simulink model "XROBO02_reference"  (R2025a)
settings: Solver=ode15s  StartTime=0  StopTime=8  MaxStep=0.002  RelTol=1e-3  AbsTol=1e-3
undefined symbols (not defined in the file): cube_l, disturbance_start, disturbance_torque_nm, F1, F2, left_target_rad, move_duration, right_target_rad, shared_payload_mass, torque_limit_scale, X, Y, Z
libraries: sm_lib x210, nesl_utility x45
(part 2 of 5)

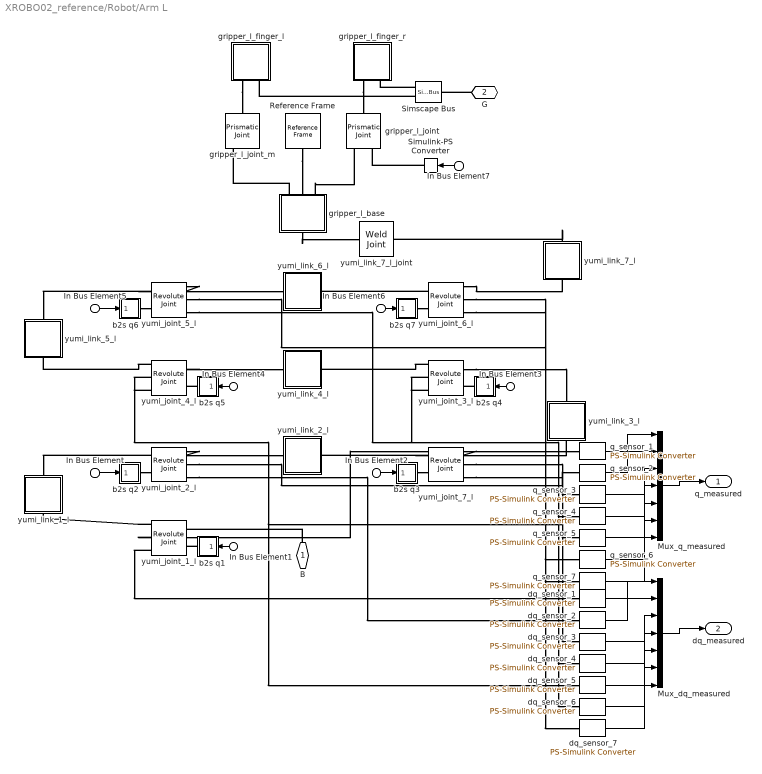
== system XROBO02_reference/Robot/Arm L ==
  In Bus Element1 : Inport  PortName=q  Element=q1
  In Bus Element : Inport  PortName=q  Element=q2
  In Bus Element2 : Inport  PortName=q  Element=q3
  In Bus Element3 : Inport  PortName=q  Element=q4
  In Bus Element4 : Inport  PortName=q  Element=q5
  In Bus Element5 : Inport  PortName=q  Element=q6
  In Bus Element6 : Inport  PortName=q  Element=q7
  In Bus Element7 : Inport  PortName=q  Element=f
  Mux_dq_measured : Mux  Inputs=7
  Mux_q_measured : Mux  Inputs=7
  Reference Frame : sm_lib/Frames and Transforms/Reference Frame
  Simscape Bus : SimscapeBus  HierarchyStrings=F1;F2
  Simulink-PS Converter : nesl_utility/Simulink-PS Converter  PhysicalDomain=network_engine_domain  SubClassName=ps_input  LeftPortType=input  RightPortType=output  PseudoPeriodic=off  Frequencies=[]  NoiseDistribution=none  NoiseParameters=[]  Unit=m  AffineConversion=off  FilteringAndDerivatives=filter  SimscapeFilterOrder=2  InputFilterTimeConstant=0.1  UdotUserProvided=0
  b2s q1 : Subsystem
  b2s q2 : Subsystem
  b2s q3 : Subsystem
  b2s q4 : Subsystem
  b2s q5 : Subsystem
  b2s q6 : Subsystem
  b2s q7 : Subsystem
  dq_sensor_{1..7} (7 alike) : nesl_utility/PS-Simulink Converter  PhysicalDomain=network_engine_domain  SubClassName=ps_output  LeftPortType=input  RightPortType=output  PseudoPeriodic=off  Frequencies=[]  VectorFormat=inherit  Unit=rad/s  AffineConversion=off
  gripper_l_base : Subsystem
  gripper_l_finger_l : Subsystem
  gripper_l_finger_r : Subsystem
  gripper_l_joint : sm_lib/Joints/Prismatic Joint  JointMode=Normal  CompositeWrenchDir=FollowerOnBase  CompositeWrenchFrame=BaseFrame  SenseConstraintForce=off  SenseConstraintTorque=off  SenseTotalForce=off  SenseTotalTorque=off  PositionTargetSpecify=off  PositionTargetPriority=High  PositionTargetValue=0  PositionTargetValueUnits=m  VelocityTargetSpecify=off  VelocityTargetPriority=High  VelocityTargetValue=0  VelocityTargetValueUnits=m/s  EquilibriumPosition=0  EquilibriumPositionUnits=m  SpringStiffness=0  SpringStiffnessUnits=N/m  DampingCoefficient=1  DampingCoefficientUnits=kg/s  LowerLimitSpecify=on  LowerLimitBound=0  LowerLimitBoundUnits=m  LowerLimitStiffness=1e6  LowerLimitStiffnessUnits=N/m  LowerLimitDamping=1e3  LowerLimitDampingUnits=N/(m/s)  LowerLimitTransitionRegionWidth=1e-4  LowerLimitTransitionRegionWidthUnits=m  UpperLimitSpecify=on  UpperLimitBound=0.025  UpperLimitBoundUnits=m  UpperLimitStiffness=1e6  UpperLimitStiffnessUnits=N/m  UpperLimitDamping=1e3  UpperLimitDampingUnits=N/(m/s)  UpperLimitTransitionRegionWidth=1e-4  UpperLimitTransitionRegionWidthUnits=m  TorqueActuationMode=ComputedTorque  MotionActuationMode=InputMotion  SensePosition=off  SenseVelocity=off  SenseAcceleration=off  SenseTorqueForce=off  SenseLowerLimitTorqueForce=off  SenseUpperLimitTorqueForce=off
  gripper_l_joint_m : sm_lib/Joints/Prismatic Joint  JointMode=Normal  CompositeWrenchDir=FollowerOnBase  CompositeWrenchFrame=BaseFrame  SenseConstraintForce=off  SenseConstraintTorque=off  SenseTotalForce=off  SenseTotalTorque=off  PositionTargetSpecify=off  PositionTargetPriority=High  PositionTargetValue=0  PositionTargetValueUnits=m  VelocityTargetSpecify=off  VelocityTargetPriority=High  VelocityTargetValue=0  VelocityTargetValueUnits=m/s  EquilibriumPosition=0  EquilibriumPositionUnits=m  SpringStiffness=0  SpringStiffnessUnits=N/m  DampingCoefficient=1  DampingCoefficientUnits=kg/s  LowerLimitSpecify=on  LowerLimitBound=0  LowerLimitBoundUnits=m  LowerLimitStiffness=1e6  LowerLimitStiffnessUnits=N/m  LowerLimitDamping=1e3  LowerLimitDampingUnits=N/(m/s)  LowerLimitTransitionRegionWidth=1e-4  LowerLimitTransitionRegionWidthUnits=m  UpperLimitSpecify=on  UpperLimitBound=0.025  UpperLimitBoundUnits=m  UpperLimitStiffness=1e6  UpperLimitStiffnessUnits=N/m  UpperLimitDamping=1e3  UpperLimitDampingUnits=N/(m/s)  UpperLimitTransitionRegionWidth=1e-4  UpperLimitTransitionRegionWidthUnits=m  TorqueActuationMode=ComputedTorque  MotionActuationMode=InputMotion  SensePosition=off  SenseVelocity=off  SenseAcceleration=off  SenseTorqueForce=off  SenseLowerLimitTorqueForce=off  SenseUpperLimitTorqueForce=off
  q_sensor_{1..7} (7 alike) : nesl_utility/PS-Simulink Converter  PhysicalDomain=network_engine_domain  SubClassName=ps_output  LeftPortType=input  RightPortType=output  PseudoPeriodic=off  Frequencies=[]  VectorFormat=inherit  Unit=rad  AffineConversion=off
  yumi_joint_1_l : sm_lib/Joints/Revolute Joint  JointMode=Normal  CompositeWrenchDir=FollowerOnBase  CompositeWrenchFrame=BaseFrame  SenseConstraintForce=off  SenseConstraintTorque=off  SenseTotalForce=off  SenseTotalTorque=off  PositionTargetSpecify=on  PositionTargetPriority=High  PositionTargetValue=0.78539816339744828  PositionTargetValueUnits=rad  VelocityTargetSpecify=on  VelocityTargetPriority=High  VelocityTargetValue=0  VelocityTargetValueUnits=rad/s  EquilibriumPosition=0  EquilibriumPositionUnits=deg  SpringStiffness=0  SpringStiffnessUnits=N*m/deg  DampingCoefficient=0.5  DampingCoefficientUnits=m^2*kg/s/rad  LowerLimitSpecify=on  LowerLimitBound=-2.94087978961  LowerLimitBoundUnits=rad  LowerLimitStiffness=1e4  LowerLimitStiffnessUnits=N*m/deg  LowerLimitDamping=10  LowerLimitDampingUnits=N*m/(deg/s)  LowerLimitTransitionRegionWidth=0.1  LowerLimitTransitionRegionWidthUnits=deg  UpperLimitSpecify=on  UpperLimitBound=2.94087978961  UpperLimitBoundUnits=rad  UpperLimitStiffness=1e4  UpperLimitStiffnessUnits=N*m/deg  UpperLimitDamping=10  UpperLimitDampingUnits=N*m/(deg/s)  UpperLimitTransitionRegionWidth=0.1  UpperLimitTransitionRegionWidthUnits=deg  TorqueActuationMode=InputTorque  MotionActuationMode=ComputedMotion  SensePosition=on  SenseVelocity=on  SenseAcceleration=off  SenseTorqueForce=off  SenseLowerLimitTorqueForce=off  SenseUpperLimitTorqueForce=off
  yumi_joint_2_l : sm_lib/Joints/Revolute Joint  JointMode=Normal  CompositeWrenchDir=FollowerOnBase  CompositeWrenchFrame=BaseFrame  SenseConstraintForce=off  SenseConstraintTorque=off  SenseTotalForce=off  SenseTotalTorque=off  PositionTargetSpecify=on  PositionTargetPriority=High  PositionTargetValue=0  PositionTargetValueUnits=rad  VelocityTargetSpecify=on  VelocityTargetPriority=High  VelocityTargetValue=0  VelocityTargetValueUnits=rad/s  EquilibriumPosition=0  EquilibriumPositionUnits=deg  SpringStiffness=0  SpringStiffnessUnits=N*m/deg  DampingCoefficient=0.5  DampingCoefficientUnits=m^2*kg/s/rad  LowerLimitSpecify=on  LowerLimitBound=-2.50454747661  LowerLimitBoundUnits=rad  LowerLimitStiffness=1e4  LowerLimitStiffnessUnits=N*m/deg  LowerLimitDamping=10  LowerLimitDampingUnits=N*m/(deg/s)  LowerLimitTransitionRegionWidth=0.1  LowerLimitTransitionRegionWidthUnits=deg  UpperLimitSpecify=on  UpperLimitBound=0.759218224618  UpperLimitBoundUnits=rad  UpperLimitStiffness=1e4  UpperLimitStiffnessUnits=N*m/deg  UpperLimitDamping=10  UpperLimitDampingUnits=N*m/(deg/s)  UpperLimitTransitionRegionWidth=0.1  UpperLimitTransitionRegionWidthUnits=deg  TorqueActuationMode=InputTorque  MotionActuationMode=ComputedMotion  SensePosition=on  SenseVelocity=on  SenseAcceleration=off  SenseTorqueForce=off  SenseLowerLimitTorqueForce=off  SenseUpperLimitTorqueForce=off
  yumi_joint_3_l : sm_lib/Joints/Revolute Joint  JointMode=Normal  CompositeWrenchDir=FollowerOnBase  CompositeWrenchFrame=BaseFrame  SenseConstraintForce=off  SenseConstraintTorque=off  SenseTotalForce=off  SenseTotalTorque=off  PositionTargetSpecify=on  PositionTargetPriority=High  PositionTargetValue=0  PositionTargetValueUnits=rad  VelocityTargetSpecify=on  VelocityTargetPriority=High  VelocityTargetValue=0  VelocityTargetValueUnits=rad/s  EquilibriumPosition=0  EquilibriumPositionUnits=deg  SpringStiffness=0  SpringStiffnessUnits=N*m/deg  DampingCoefficient=0.5  DampingCoefficientUnits=m^2*kg/s/rad  LowerLimitSpecify=on  LowerLimitBound=-2.15548162621  LowerLimitBoundUnits=rad  LowerLimitStiffness=1e4  LowerLimitStiffnessUnits=N*m/deg  LowerLimitDamping=10  LowerLimitDampingUnits=N*m/(deg/s)  LowerLimitTransitionRegionWidth=0.1  LowerLimitTransitionRegionWidthUnits=deg  UpperLimitSpecify=on  UpperLimitBound=1.3962634016  UpperLimitBoundUnits=rad  UpperLimitStiffness=1e4  UpperLimitStiffnessUnits=N*m/deg  UpperLimitDamping=10  UpperLimitDampingUnits=N*m/(deg/s)  UpperLimitTransitionRegionWidth=0.1  UpperLimitTransitionRegionWidthUnits=deg  TorqueActuationMode=InputTorque  MotionActuationMode=ComputedMotion  SensePosition=on  SenseVelocity=on  SenseAcceleration=off  SenseTorqueForce=off  SenseLowerLimitTorqueForce=off  SenseUpperLimitTorqueForce=off
  yumi_joint_4_l : sm_lib/Joints/Revolute Joint  JointMode=Normal  CompositeWrenchDir=FollowerOnBase  CompositeWrenchFrame=BaseFrame  SenseConstraintForce=off  SenseConstraintTorque=off  SenseTotalForce=off  SenseTotalTorque=off  PositionTargetSpecify=on  PositionTargetPriority=High  PositionTargetValue=0  PositionTargetValueUnits=rad  VelocityTargetSpecify=on  VelocityTargetPriority=High  VelocityTargetValue=0  VelocityTargetValueUnits=rad/s  EquilibriumPosition=0  EquilibriumPositionUnits=deg  SpringStiffness=0  SpringStiffnessUnits=N*m/deg  DampingCoefficient=0.5  DampingCoefficientUnits=m^2*kg/s/rad  LowerLimitSpecify=on  LowerLimitBound=-5.06145483078  LowerLimitBoundUnits=rad  LowerLimitStiffness=1e4  LowerLimitStiffnessUnits=N*m/deg  LowerLimitDamping=10  LowerLimitDampingUnits=N*m/(deg/s)  LowerLimitTransitionRegionWidth=0.1  LowerLimitTransitionRegionWidthUnits=deg  UpperLimitSpecify=on  UpperLimitBound=5.06145483078  UpperLimitBoundUnits=rad  UpperLimitStiffness=1e4  UpperLimitStiffnessUnits=N*m/deg  UpperLimitDamping=10  UpperLimitDampingUnits=N*m/(deg/s)  UpperLimitTransitionRegionWidth=0.1  UpperLimitTransitionRegionWidthUnits=deg  TorqueActuationMode=InputTorque  MotionActuationMode=ComputedMotion  SensePosition=on  SenseVelocity=on  SenseAcceleration=off  SenseTorqueForce=off  SenseLowerLimitTorqueForce=off  SenseUpperLimitTorqueForce=off
  yumi_joint_5_l : sm_lib/Joints/Revolute Joint  JointMode=Normal  CompositeWrenchDir=FollowerOnBase  CompositeWrenchFrame=BaseFrame  SenseConstraintForce=off  SenseConstraintTorque=off  SenseTotalForce=off  SenseTotalTorque=off  PositionTargetSpecify=on  PositionTargetPriority=High  PositionTargetValue=0  PositionTargetValueUnits=rad  VelocityTargetSpecify=on  VelocityTargetPriority=High  VelocityTargetValue=0  VelocityTargetValueUnits=rad/s  EquilibriumPosition=0  EquilibriumPositionUnits=deg  SpringStiffness=0  SpringStiffnessUnits=N*m/deg  DampingCoefficient=0.5  DampingCoefficientUnits=m^2*kg/s/rad  LowerLimitSpecify=on  LowerLimitBound=-1.53588974176  LowerLimitBoundUnits=rad  LowerLimitStiffness=1e4  LowerLimitStiffnessUnits=N*m/deg  LowerLimitDamping=10  LowerLimitDampingUnits=N*m/(deg/s)  LowerLimitTransitionRegionWidth=0.1  LowerLimitTransitionRegionWidthUnits=deg  UpperLimitSpecify=on  UpperLimitBound=2.40855436775  UpperLimitBoundUnits=rad  UpperLimitStiffness=1e4  UpperLimitStiffnessUnits=N*m/deg  UpperLimitDamping=10  UpperLimitDampingUnits=N*m/(deg/s)  UpperLimitTransitionRegionWidth=0.1  UpperLimitTransitionRegionWidthUnits=deg  TorqueActuationMode=InputTorque  MotionActuationMode=ComputedMotion  SensePosition=on  SenseVelocity=on  SenseAcceleration=off  SenseTorqueForce=off  SenseLowerLimitTorqueForce=off  SenseUpperLimitTorqueForce=off
  yumi_joint_6_l : sm_lib/Joints/Revolute Joint  JointMode=Normal  CompositeWrenchDir=FollowerOnBase  CompositeWrenchFrame=BaseFrame  SenseConstraintForce=off  SenseConstraintTorque=off  SenseTotalForce=off  SenseTotalTorque=off  PositionTargetSpecify=on  PositionTargetPriority=High  PositionTargetValue=0  PositionTargetValueUnits=rad  VelocityTargetSpecify=on  VelocityTargetPriority=High  VelocityTargetValue=0  VelocityTargetValueUnits=rad/s  EquilibriumPosition=0  EquilibriumPositionUnits=deg  SpringStiffness=0  SpringStiffnessUnits=N*m/deg  DampingCoefficient=0.5  DampingCoefficientUnits=m^2*kg/s/rad  LowerLimitSpecify=on  LowerLimitBound=-3.99680398707  LowerLimitBoundUnits=rad  LowerLimitStiffness=1e4  LowerLimitStiffnessUnits=N*m/deg  LowerLimitDamping=10  LowerLimitDampingUnits=N*m/(deg/s)  LowerLimitTransitionRegionWidth=0.1  LowerLimitTransitionRegionWidthUnits=deg  UpperLimitSpecify=on  UpperLimitBound=3.99680398707  UpperLimitBoundUnits=rad  UpperLimitStiffness=1e4  UpperLimitStiffnessUnits=N*m/deg  UpperLimitDamping=10  UpperLimitDampingUnits=N*m/(deg/s)  UpperLimitTransitionRegionWidth=0.1  UpperLimitTransitionRegionWidthUnits=deg  TorqueActuationMode=InputTorque  MotionActuationMode=ComputedMotion  SensePosition=on  SenseVelocity=on  SenseAcceleration=off  SenseTorqueForce=off  SenseLowerLimitTorqueForce=off  SenseUpperLimitTorqueForce=off
  yumi_joint_7_l : sm_lib/Joints/Revolute Joint  JointMode=Normal  CompositeWrenchDir=FollowerOnBase  CompositeWrenchFrame=BaseFrame  SenseConstraintForce=off  SenseConstraintTorque=off  SenseTotalForce=off  SenseTotalTorque=off  PositionTargetSpecify=on  PositionTargetPriority=High  PositionTargetValue=0  PositionTargetValueUnits=rad  VelocityTargetSpecify=on  VelocityTargetPriority=High  VelocityTargetValue=0  VelocityTargetValueUnits=rad/s  EquilibriumPosition=0  EquilibriumPositionUnits=deg  SpringStiffness=0  SpringStiffnessUnits=N*m/deg  DampingCoefficient=0.5  DampingCoefficientUnits=m^2*kg/s/rad  LowerLimitSpecify=on  LowerLimitBound=-2.94087978961  LowerLimitBoundUnits=rad  LowerLimitStiffness=1e4  LowerLimitStiffnessUnits=N*m/deg  LowerLimitDamping=10  LowerLimitDampingUnits=N*m/(deg/s)  LowerLimitTransitionRegionWidth=0.1  LowerLimitTransitionRegionWidthUnits=deg  UpperLimitSpecify=on  UpperLimitBound=2.94087978961  UpperLimitBoundUnits=rad  UpperLimitStiffness=1e4  UpperLimitStiffnessUnits=N*m/deg  UpperLimitDamping=10  UpperLimitDampingUnits=N*m/(deg/s)  UpperLimitTransitionRegionWidth=0.1  UpperLimitTransitionRegionWidthUnits=deg  TorqueActuationMode=InputTorque  MotionActuationMode=ComputedMotion  SensePosition=on  SenseVelocity=on  SenseAcceleration=off  SenseTorqueForce=off  SenseLowerLimitTorqueForce=off  SenseUpperLimitTorqueForce=off
  yumi_link_1_l : Subsystem
  yumi_link_2_l : Subsystem
  yumi_link_3_l : Subsystem
  yumi_link_4_l : Subsystem
  yumi_link_5_l : Subsystem
  yumi_link_6_l : Subsystem
  yumi_link_7_l : Subsystem
  yumi_link_7_l_joint : sm_lib/Joints/Weld Joint  JointMode=Normal  CompositeWrenchDir=FollowerOnBase  CompositeWrenchFrame=BaseFrame  SenseConstraintForce=off  SenseConstraintTorque=off  SenseTotalForce=off  SenseTotalTorque=off
  B : PMIOPort  Side=Right
  G : PMIOPort  Port=2  Side=Right
  q_measured : Outport
  dq_measured : Outport  Port=2
  wires:
  In Bus Element7/1 -> Simulink-PS Converter/1
  In Bus Element1/1 -> b2s q1/1(tau)
  In Bus Element/1 -> b2s q2/1(tau)
  In Bus Element2/1 -> b2s q3/1(tau)
  In Bus Element3/1 -> b2s q4/1(tau)
  In Bus Element4/1 -> b2s q5/1(tau)
  In Bus Element5/1 -> b2s q6/1(tau)
  In Bus Element6/1 -> b2s q7/1(tau)
  q_sensor_1/1 -> Mux_q_measured/1
  dq_sensor_1/1 -> Mux_dq_measured/1
  q_sensor_2/1 -> Mux_q_measured/2
  dq_sensor_2/1 -> Mux_dq_measured/2
  q_sensor_3/1 -> Mux_q_measured/3
  dq_sensor_3/1 -> Mux_dq_measured/3
  q_sensor_4/1 -> Mux_q_measured/4
  dq_sensor_4/1 -> Mux_dq_measured/4
  q_sensor_5/1 -> Mux_q_measured/5
  dq_sensor_5/1 -> Mux_dq_measured/5
  q_sensor_6/1 -> Mux_q_measured/6
  dq_sensor_6/1 -> Mux_dq_measured/6
  q_sensor_7/1 -> Mux_q_measured/7
  dq_sensor_7/1 -> Mux_dq_measured/7
  Mux_q_measured/1 -> q_measured/1
  Mux_dq_measured/1 -> dq_measured/1
  connections:
  gripper_l_base/LConn1 -- yumi_link_7_l_joint/RConn1
  gripper_l_finger_l/LConn1 -- gripper_l_joint_m/RConn1
  gripper_l_base/RConn3 -- gripper_l_joint/LConn1
  yumi_joint_1_l/RConn1 -- yumi_link_1_l/LConn1
  yumi_joint_2_l/LConn1 -- yumi_link_1_l/RConn1
  yumi_joint_4_l/RConn1 -- yumi_link_5_l/LConn1
  yumi_link_7_l/RConn1 -- yumi_link_7_l_joint/LConn1
  yumi_joint_4_l/LConn1 -- yumi_link_4_l/RConn1
  yumi_joint_7_l/RConn1 -- yumi_link_3_l/LConn1
  yumi_joint_3_l/RConn1 -- yumi_link_4_l/LConn1
  yumi_joint_2_l/RConn1 -- yumi_link_2_l/LConn1
  yumi_joint_5_l/LConn1 -- yumi_link_5_l/RConn1
  yumi_joint_6_l/LConn1 -- yumi_link_6_l/RConn1
  yumi_joint_5_l/RConn1 -- yumi_link_6_l/LConn1
  gripper_l_base/RConn1 -- gripper_l_joint_m/LConn1
  yumi_joint_3_l/LConn1 -- yumi_link_3_l/RConn1
  gripper_l_finger_r/LConn1 -- gripper_l_joint/RConn1
  yumi_joint_7_l/LConn1 -- yumi_link_2_l/RConn1
  yumi_joint_6_l/RConn1 -- yumi_link_7_l/LConn1
  B/RConn1 -- yumi_joint_1_l/LConn1
  Reference Frame/RConn1 -- gripper_l_base/RConn2
  G/RConn1 -- Simscape Bus/RConn1
  Simscape Bus/LConn1 -- gripper_l_finger_r/LConn2
  Simscape Bus/LConn2 -- gripper_l_finger_l/LConn2
  b2s q1/RConn1 -- yumi_joint_1_l/LConn2
  b2s q2/RConn1 -- yumi_joint_2_l/LConn2
  b2s q3/RConn1 -- yumi_joint_7_l/LConn2
  b2s q4/RConn1 -- yumi_joint_3_l/LConn2
  b2s q5/RConn1 -- yumi_joint_4_l/LConn2
  b2s q6/RConn1 -- yumi_joint_5_l/LConn2
  b2s q7/RConn1 -- yumi_joint_6_l/LConn2
  yumi_joint_1_l/RConn2 -- q_sensor_1/LConn1
  yumi_joint_1_l/RConn3 -- dq_sensor_1/LConn1
  yumi_joint_2_l/RConn2 -- q_sensor_2/LConn1
  yumi_joint_2_l/RConn3 -- dq_sensor_2/LConn1
  yumi_joint_7_l/RConn2 -- q_sensor_3/LConn1
  yumi_joint_7_l/RConn3 -- dq_sensor_3/LConn1
  yumi_joint_3_l/RConn2 -- q_sensor_4/LConn1
  yumi_joint_3_l/RConn3 -- dq_sensor_4/LConn1
  yumi_joint_4_l/RConn2 -- q_sensor_5/LConn1
  yumi_joint_4_l/RConn3 -- dq_sensor_5/LConn1
  yumi_joint_5_l/RConn2 -- q_sensor_6/LConn1
  yumi_joint_5_l/RConn3 -- dq_sensor_6/LConn1
  yumi_joint_6_l/RConn2 -- q_sensor_7/LConn1
  yumi_joint_6_l/RConn3 -- dq_sensor_7/LConn1
  Simulink-PS Converter/RConn1 -- gripper_l_joint/LConn2

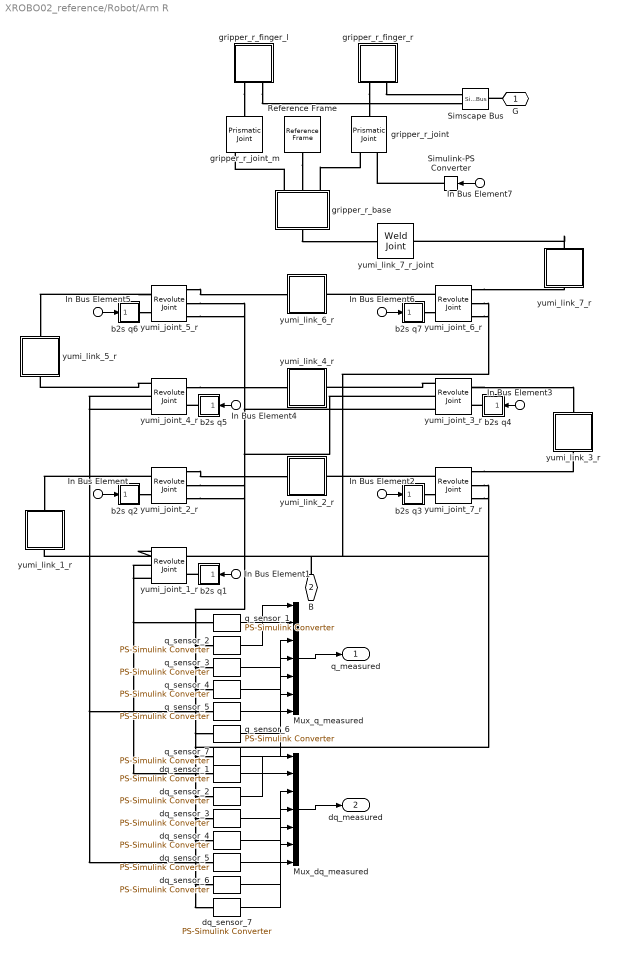
== system XROBO02_reference/Robot/Arm R ==
  In Bus Element1 : Inport  PortName=q  Element=q1
  In Bus Element : Inport  PortName=q  Element=q2
  In Bus Element2 : Inport  PortName=q  Element=q3
  In Bus Element3 : Inport  PortName=q  Element=q4
  In Bus Element4 : Inport  PortName=q  Element=q5
  In Bus Element5 : Inport  PortName=q  Element=q6
  In Bus Element6 : Inport  PortName=q  Element=q7
  In Bus Element7 : Inport  PortName=q  Element=f
  Mux_dq_measured : Mux  Inputs=7
  Mux_q_measured : Mux  Inputs=7
  Reference Frame : sm_lib/Frames and Transforms/Reference Frame
  Simscape Bus : SimscapeBus  HierarchyStrings=F1;F2
  Simulink-PS Converter : nesl_utility/Simulink-PS Converter  PhysicalDomain=network_engine_domain  SubClassName=ps_input  LeftPortType=input  RightPortType=output  PseudoPeriodic=off  Frequencies=[]  NoiseDistribution=none  NoiseParameters=[]  Unit=m  AffineConversion=off  FilteringAndDerivatives=filter  SimscapeFilterOrder=2  InputFilterTimeConstant=0.1  UdotUserProvided=0
  b2s q1 : Subsystem
  b2s q2 : Subsystem
  b2s q3 : Subsystem
  b2s q4 : Subsystem
  b2s q5 : Subsystem
  b2s q6 : Subsystem
  b2s q7 : Subsystem
  dq_sensor_{1..7} (7 alike) : nesl_utility/PS-Simulink Converter  PhysicalDomain=network_engine_domain  SubClassName=ps_output  LeftPortType=input  RightPortType=output  PseudoPeriodic=off  Frequencies=[]  VectorFormat=inherit  Unit=rad/s  AffineConversion=off
  gripper_r_base : Subsystem
  gripper_r_finger_l : Subsystem
  gripper_r_finger_r : Subsystem
  gripper_r_joint : sm_lib/Joints/Prismatic Joint  JointMode=Normal  CompositeWrenchDir=FollowerOnBase  CompositeWrenchFrame=BaseFrame  SenseConstraintForce=off  SenseConstraintTorque=off  SenseTotalForce=off  SenseTotalTorque=off  PositionTargetSpecify=off  PositionTargetPriority=High  PositionTargetValue=0  PositionTargetValueUnits=m  VelocityTargetSpecify=off  VelocityTargetPriority=High  VelocityTargetValue=0  VelocityTargetValueUnits=m/s  EquilibriumPosition=0  EquilibriumPositionUnits=m  SpringStiffness=0  SpringStiffnessUnits=N/m  DampingCoefficient=1  DampingCoefficientUnits=kg/s  LowerLimitSpecify=on  LowerLimitBound=0  LowerLimitBoundUnits=m  LowerLimitStiffness=1e6  LowerLimitStiffnessUnits=N/m  LowerLimitDamping=1e3  LowerLimitDampingUnits=N/(m/s)  LowerLimitTransitionRegionWidth=1e-4  LowerLimitTransitionRegionWidthUnits=m  UpperLimitSpecify=on  UpperLimitBound=0.025  UpperLimitBoundUnits=m  UpperLimitStiffness=1e6  UpperLimitStiffnessUnits=N/m  UpperLimitDamping=1e3  UpperLimitDampingUnits=N/(m/s)  UpperLimitTransitionRegionWidth=1e-4  UpperLimitTransitionRegionWidthUnits=m  TorqueActuationMode=ComputedTorque  MotionActuationMode=InputMotion  SensePosition=off  SenseVelocity=off  SenseAcceleration=off  SenseTorqueForce=off  SenseLowerLimitTorqueForce=off  SenseUpperLimitTorqueForce=off
  gripper_r_joint_m : sm_lib/Joints/Prismatic Joint  JointMode=Normal  CompositeWrenchDir=FollowerOnBase  CompositeWrenchFrame=BaseFrame  SenseConstraintForce=off  SenseConstraintTorque=off  SenseTotalForce=off  SenseTotalTorque=off  PositionTargetSpecify=off  PositionTargetPriority=High  PositionTargetValue=0  PositionTargetValueUnits=m  VelocityTargetSpecify=off  VelocityTargetPriority=High  VelocityTargetValue=0  VelocityTargetValueUnits=m/s  EquilibriumPosition=0  EquilibriumPositionUnits=m  SpringStiffness=0  SpringStiffnessUnits=N/m  DampingCoefficient=1  DampingCoefficientUnits=kg/s  LowerLimitSpecify=on  LowerLimitBound=0  LowerLimitBoundUnits=m  LowerLimitStiffness=1e6  LowerLimitStiffnessUnits=N/m  LowerLimitDamping=1e3  LowerLimitDampingUnits=N/(m/s)  LowerLimitTransitionRegionWidth=1e-4  LowerLimitTransitionRegionWidthUnits=m  UpperLimitSpecify=on  UpperLimitBound=0.025  UpperLimitBoundUnits=m  UpperLimitStiffness=1e6  UpperLimitStiffnessUnits=N/m  UpperLimitDamping=1e3  UpperLimitDampingUnits=N/(m/s)  UpperLimitTransitionRegionWidth=1e-4  UpperLimitTransitionRegionWidthUnits=m  TorqueActuationMode=ComputedTorque  MotionActuationMode=InputMotion  SensePosition=off  SenseVelocity=off  SenseAcceleration=off  SenseTorqueForce=off  SenseLowerLimitTorqueForce=off  SenseUpperLimitTorqueForce=off
  q_sensor_{1..7} (7 alike) : nesl_utility/PS-Simulink Converter  PhysicalDomain=network_engine_domain  SubClassName=ps_output  LeftPortType=input  RightPortType=output  PseudoPeriodic=off  Frequencies=[]  VectorFormat=inherit  Unit=rad  AffineConversion=off
  yumi_joint_1_r : sm_lib/Joints/Revolute Joint  JointMode=Normal  CompositeWrenchDir=FollowerOnBase  CompositeWrenchFrame=BaseFrame  SenseConstraintForce=off  SenseConstraintTorque=off  SenseTotalForce=off  SenseTotalTorque=off  PositionTargetSpecify=on  PositionTargetPriority=High  PositionTargetValue=-0.78539816339744828  PositionTargetValueUnits=rad  VelocityTargetSpecify=on  VelocityTargetPriority=High  VelocityTargetValue=0  VelocityTargetValueUnits=rad/s  EquilibriumPosition=0  EquilibriumPositionUnits=deg  SpringStiffness=0  SpringStiffnessUnits=N*m/deg  DampingCoefficient=0.5  DampingCoefficientUnits=m^2*kg/s/rad  LowerLimitSpecify=on  LowerLimitBound=-2.94087978961  LowerLimitBoundUnits=rad  LowerLimitStiffness=1e4  LowerLimitStiffnessUnits=N*m/deg  LowerLimitDamping=10  LowerLimitDampingUnits=N*m/(deg/s)  LowerLimitTransitionRegionWidth=0.1  LowerLimitTransitionRegionWidthUnits=deg  UpperLimitSpecify=on  UpperLimitBound=2.94087978961  UpperLimitBoundUnits=rad  UpperLimitStiffness=1e4  UpperLimitStiffnessUnits=N*m/deg  UpperLimitDamping=10  UpperLimitDampingUnits=N*m/(deg/s)  UpperLimitTransitionRegionWidth=0.1  UpperLimitTransitionRegionWidthUnits=deg  TorqueActuationMode=InputTorque  MotionActuationMode=ComputedMotion  SensePosition=on  SenseVelocity=on  SenseAcceleration=off  SenseTorqueForce=off  SenseLowerLimitTorqueForce=off  SenseUpperLimitTorqueForce=off
  yumi_joint_2_r : sm_lib/Joints/Revolute Joint  JointMode=Normal  CompositeWrenchDir=FollowerOnBase  CompositeWrenchFrame=BaseFrame  SenseConstraintForce=off  SenseConstraintTorque=off  SenseTotalForce=off  SenseTotalTorque=off  PositionTargetSpecify=on  PositionTargetPriority=High  PositionTargetValue=0  PositionTargetValueUnits=rad  VelocityTargetSpecify=on  VelocityTargetPriority=High  VelocityTargetValue=0  VelocityTargetValueUnits=rad/s  EquilibriumPosition=0  EquilibriumPositionUnits=deg  SpringStiffness=0  SpringStiffnessUnits=N*m/deg  DampingCoefficient=0.5  DampingCoefficientUnits=m^2*kg/s/rad  LowerLimitSpecify=on  LowerLimitBound=-2.50454747661  LowerLimitBoundUnits=rad  LowerLimitStiffness=1e4  LowerLimitStiffnessUnits=N*m/deg  LowerLimitDamping=10  LowerLimitDampingUnits=N*m/(deg/s)  LowerLimitTransitionRegionWidth=0.1  LowerLimitTransitionRegionWidthUnits=deg  UpperLimitSpecify=on  UpperLimitBound=0.759218224618  UpperLimitBoundUnits=rad  UpperLimitStiffness=1e4  UpperLimitStiffnessUnits=N*m/deg  UpperLimitDamping=10  UpperLimitDampingUnits=N*m/(deg/s)  UpperLimitTransitionRegionWidth=0.1  UpperLimitTransitionRegionWidthUnits=deg  TorqueActuationMode=InputTorque  MotionActuationMode=ComputedMotion  SensePosition=on  SenseVelocity=on  SenseAcceleration=off  SenseTorqueForce=off  SenseLowerLimitTorqueForce=off  SenseUpperLimitTorqueForce=off
  yumi_joint_3_r : sm_lib/Joints/Revolute Joint  JointMode=Normal  CompositeWrenchDir=FollowerOnBase  CompositeWrenchFrame=BaseFrame  SenseConstraintForce=off  SenseConstraintTorque=off  SenseTotalForce=off  SenseTotalTorque=off  PositionTargetSpecify=on  PositionTargetPriority=High  PositionTargetValue=0  PositionTargetValueUnits=rad  VelocityTargetSpecify=on  VelocityTargetPriority=High  VelocityTargetValue=0  VelocityTargetValueUnits=rad/s  EquilibriumPosition=0  EquilibriumPositionUnits=deg  SpringStiffness=0  SpringStiffnessUnits=N*m/deg  DampingCoefficient=0.5  DampingCoefficientUnits=m^2*kg/s/rad  LowerLimitSpecify=on  LowerLimitBound=-2.15548162621  LowerLimitBoundUnits=rad  LowerLimitStiffness=1e4  LowerLimitStiffnessUnits=N*m/deg  LowerLimitDamping=10  LowerLimitDampingUnits=N*m/(deg/s)  LowerLimitTransitionRegionWidth=0.1  LowerLimitTransitionRegionWidthUnits=deg  UpperLimitSpecify=on  UpperLimitBound=1.3962634016  UpperLimitBoundUnits=rad  UpperLimitStiffness=1e4  UpperLimitStiffnessUnits=N*m/deg  UpperLimitDamping=10  UpperLimitDampingUnits=N*m/(deg/s)  UpperLimitTransitionRegionWidth=0.1  UpperLimitTransitionRegionWidthUnits=deg  TorqueActuationMode=InputTorque  MotionActuationMode=ComputedMotion  SensePosition=on  SenseVelocity=on  SenseAcceleration=off  SenseTorqueForce=off  SenseLowerLimitTorqueForce=off  SenseUpperLimitTorqueForce=off
  yumi_joint_4_r : sm_lib/Joints/Revolute Joint  JointMode=Normal  CompositeWrenchDir=FollowerOnBase  CompositeWrenchFrame=BaseFrame  SenseConstraintForce=off  SenseConstraintTorque=off  SenseTotalForce=off  SenseTotalTorque=off  PositionTargetSpecify=on  PositionTargetPriority=High  PositionTargetValue=0  PositionTargetValueUnits=rad  VelocityTargetSpecify=on  VelocityTargetPriority=High  VelocityTargetValue=0  VelocityTargetValueUnits=rad/s  EquilibriumPosition=0  EquilibriumPositionUnits=deg  SpringStiffness=0  SpringStiffnessUnits=N*m/deg  DampingCoefficient=0.5  DampingCoefficientUnits=m^2*kg/s/rad  LowerLimitSpecify=on  LowerLimitBound=-5.06145483078  LowerLimitBoundUnits=rad  LowerLimitStiffness=1e4  LowerLimitStiffnessUnits=N*m/deg  LowerLimitDamping=10  LowerLimitDampingUnits=N*m/(deg/s)  LowerLimitTransitionRegionWidth=0.1  LowerLimitTransitionRegionWidthUnits=deg  UpperLimitSpecify=on  UpperLimitBound=5.06145483078  UpperLimitBoundUnits=rad  UpperLimitStiffness=1e4  UpperLimitStiffnessUnits=N*m/deg  UpperLimitDamping=10  UpperLimitDampingUnits=N*m/(deg/s)  UpperLimitTransitionRegionWidth=0.1  UpperLimitTransitionRegionWidthUnits=deg  TorqueActuationMode=InputTorque  MotionActuationMode=ComputedMotion  SensePosition=on  SenseVelocity=on  SenseAcceleration=off  SenseTorqueForce=off  SenseLowerLimitTorqueForce=off  SenseUpperLimitTorqueForce=off
  yumi_joint_5_r : sm_lib/Joints/Revolute Joint  JointMode=Normal  CompositeWrenchDir=FollowerOnBase  CompositeWrenchFrame=BaseFrame  SenseConstraintForce=off  SenseConstraintTorque=off  SenseTotalForce=off  SenseTotalTorque=off  PositionTargetSpecify=on  PositionTargetPriority=High  PositionTargetValue=0  PositionTargetValueUnits=rad  VelocityTargetSpecify=on  VelocityTargetPriority=High  VelocityTargetValue=0  VelocityTargetValueUnits=rad/s  EquilibriumPosition=0  EquilibriumPositionUnits=deg  SpringStiffness=0  SpringStiffnessUnits=N*m/deg  DampingCoefficient=0.5  DampingCoefficientUnits=m^2*kg/s/rad  LowerLimitSpecify=on  LowerLimitBound=-1.53588974176  LowerLimitBoundUnits=rad  LowerLimitStiffness=1e4  LowerLimitStiffnessUnits=N*m/deg  LowerLimitDamping=10  LowerLimitDampingUnits=N*m/(deg/s)  LowerLimitTransitionRegionWidth=0.1  LowerLimitTransitionRegionWidthUnits=deg  UpperLimitSpecify=on  UpperLimitBound=2.40855436775  UpperLimitBoundUnits=rad  UpperLimitStiffness=1e4  UpperLimitStiffnessUnits=N*m/deg  UpperLimitDamping=10  UpperLimitDampingUnits=N*m/(deg/s)  UpperLimitTransitionRegionWidth=0.1  UpperLimitTransitionRegionWidthUnits=deg  TorqueActuationMode=InputTorque  MotionActuationMode=ComputedMotion  SensePosition=on  SenseVelocity=on  SenseAcceleration=off  SenseTorqueForce=off  SenseLowerLimitTorqueForce=off  SenseUpperLimitTorqueForce=off
  yumi_joint_6_r : sm_lib/Joints/Revolute Joint  JointMode=Normal  CompositeWrenchDir=FollowerOnBase  CompositeWrenchFrame=BaseFrame  SenseConstraintForce=off  SenseConstraintTorque=off  SenseTotalForce=off  SenseTotalTorque=off  PositionTargetSpecify=on  PositionTargetPriority=High  PositionTargetValue=0  PositionTargetValueUnits=rad  VelocityTargetSpecify=on  VelocityTargetPriority=High  VelocityTargetValue=0  VelocityTargetValueUnits=rad/s  EquilibriumPosition=0  EquilibriumPositionUnits=deg  SpringStiffness=0  SpringStiffnessUnits=N*m/deg  DampingCoefficient=0.5  DampingCoefficientUnits=m^2*kg/s/rad  LowerLimitSpecify=on  LowerLimitBound=-3.99680398707  LowerLimitBoundUnits=rad  LowerLimitStiffness=1e4  LowerLimitStiffnessUnits=N*m/deg  LowerLimitDamping=10  LowerLimitDampingUnits=N*m/(deg/s)  LowerLimitTransitionRegionWidth=0.1  LowerLimitTransitionRegionWidthUnits=deg  UpperLimitSpecify=on  UpperLimitBound=3.99680398707  UpperLimitBoundUnits=rad  UpperLimitStiffness=1e4  UpperLimitStiffnessUnits=N*m/deg  UpperLimitDamping=10  UpperLimitDampingUnits=N*m/(deg/s)  UpperLimitTransitionRegionWidth=0.1  UpperLimitTransitionRegionWidthUnits=deg  TorqueActuationMode=InputTorque  MotionActuationMode=ComputedMotion  SensePosition=on  SenseVelocity=on  SenseAcceleration=off  SenseTorqueForce=off  SenseLowerLimitTorqueForce=off  SenseUpperLimitTorqueForce=off
  yumi_joint_7_r : sm_lib/Joints/Revolute Joint  JointMode=Normal  CompositeWrenchDir=FollowerOnBase  CompositeWrenchFrame=BaseFrame  SenseConstraintForce=off  SenseConstraintTorque=off  SenseTotalForce=off  SenseTotalTorque=off  PositionTargetSpecify=on  PositionTargetPriority=High  PositionTargetValue=0  PositionTargetValueUnits=rad  VelocityTargetSpecify=on  VelocityTargetPriority=High  VelocityTargetValue=0  VelocityTargetValueUnits=rad/s  EquilibriumPosition=0  EquilibriumPositionUnits=deg  SpringStiffness=0  SpringStiffnessUnits=N*m/deg  DampingCoefficient=0.5  DampingCoefficientUnits=m^2*kg/s/rad  LowerLimitSpecify=on  LowerLimitBound=-2.94087978961  LowerLimitBoundUnits=rad  LowerLimitStiffness=1e4  LowerLimitStiffnessUnits=N*m/deg  LowerLimitDamping=10  LowerLimitDampingUnits=N*m/(deg/s)  LowerLimitTransitionRegionWidth=0.1  LowerLimitTransitionRegionWidthUnits=deg  UpperLimitSpecify=on  UpperLimitBound=2.94087978961  UpperLimitBoundUnits=rad  UpperLimitStiffness=1e4  UpperLimitStiffnessUnits=N*m/deg  UpperLimitDamping=10  UpperLimitDampingUnits=N*m/(deg/s)  UpperLimitTransitionRegionWidth=0.1  UpperLimitTransitionRegionWidthUnits=deg  TorqueActuationMode=InputTorque  MotionActuationMode=ComputedMotion  SensePosition=on  SenseVelocity=on  SenseAcceleration=off  SenseTorqueForce=off  SenseLowerLimitTorqueForce=off  SenseUpperLimitTorqueForce=off
  yumi_link_1_r : Subsystem
  yumi_link_2_r : Subsystem
  yumi_link_3_r : Subsystem
  yumi_link_4_r : Subsystem
  yumi_link_5_r : Subsystem
  yumi_link_6_r : Subsystem
  yumi_link_7_r : Subsystem
  yumi_link_7_r_joint : sm_lib/Joints/Weld Joint  JointMode=Normal  CompositeWrenchDir=FollowerOnBase  CompositeWrenchFrame=BaseFrame  SenseConstraintForce=off  SenseConstraintTorque=off  SenseTotalForce=off  SenseTotalTorque=off
  G : PMIOPort  Side=Right
  B : PMIOPort  Port=2  Side=Right
  q_measured : Outport
  dq_measured : Outport  Port=2
  wires:
  In Bus Element7/1 -> Simulink-PS Converter/1
  In Bus Element1/1 -> b2s q1/1(tau)
  In Bus Element/1 -> b2s q2/1(tau)
  In Bus Element2/1 -> b2s q3/1(tau)
  In Bus Element3/1 -> b2s q4/1(tau)
  In Bus Element4/1 -> b2s q5/1(tau)
  In Bus Element5/1 -> b2s q6/1(tau)
  In Bus Element6/1 -> b2s q7/1(tau)
  q_sensor_1/1 -> Mux_q_measured/1
  dq_sensor_1/1 -> Mux_dq_measured/1
  q_sensor_2/1 -> Mux_q_measured/2
  dq_sensor_2/1 -> Mux_dq_measured/2
  q_sensor_3/1 -> Mux_q_measured/3
  dq_sensor_3/1 -> Mux_dq_measured/3
  q_sensor_4/1 -> Mux_q_measured/4
  dq_sensor_4/1 -> Mux_dq_measured/4
  q_sensor_5/1 -> Mux_q_measured/5
  dq_sensor_5/1 -> Mux_dq_measured/5
  q_sensor_6/1 -> Mux_q_measured/6
  dq_sensor_6/1 -> Mux_dq_measured/6
  q_sensor_7/1 -> Mux_q_measured/7
  dq_sensor_7/1 -> Mux_dq_measured/7
  Mux_q_measured/1 -> q_measured/1
  Mux_dq_measured/1 -> dq_measured/1
  connections:
  yumi_joint_1_r/RConn1 -- yumi_link_1_r/LConn1
  gripper_r_finger_l/LConn1 -- gripper_r_joint_m/RConn1
  yumi_joint_2_r/RConn1 -- yumi_link_2_r/LConn1
  yumi_joint_6_r/RConn1 -- yumi_link_7_r/LConn1
  yumi_joint_2_r/LConn1 -- yumi_link_1_r/RConn1
  yumi_joint_5_r/LConn1 -- yumi_link_5_r/RConn1
  yumi_joint_4_r/RConn1 -- yumi_link_5_r/LConn1
  yumi_joint_3_r/LConn1 -- yumi_link_3_r/RConn1
  yumi_joint_3_r/RConn1 -- yumi_link_4_r/LConn1
  yumi_joint_5_r/RConn1 -- yumi_link_6_r/LConn1
  yumi_joint_7_r/RConn1 -- yumi_link_3_r/LConn1
  yumi_joint_7_r/LConn1 -- yumi_link_2_r/RConn1
  yumi_joint_4_r/LConn1 -- yumi_link_4_r/RConn1
  yumi_joint_6_r/LConn1 -- yumi_link_6_r/RConn1
  gripper_r_base/LConn1 -- yumi_link_7_r_joint/RConn1
  yumi_link_7_r/RConn1 -- yumi_link_7_r_joint/LConn1
  gripper_r_base/RConn1 -- gripper_r_joint_m/LConn1
  gripper_r_base/RConn3 -- gripper_r_joint/LConn1
  gripper_r_finger_r/LConn1 -- gripper_r_joint/RConn1
  B/RConn1 -- yumi_joint_1_r/LConn1
  Reference Frame/RConn1 -- gripper_r_base/RConn2
  G/RConn1 -- Simscape Bus/RConn1
  gripper_r_finger_r/LConn2 -- Simscape Bus/LConn1
  gripper_r_finger_l/LConn2 -- Simscape Bus/LConn2
  b2s q1/RConn1 -- yumi_joint_1_r/LConn2
  b2s q2/RConn1 -- yumi_joint_2_r/LConn2
  b2s q3/RConn1 -- yumi_joint_7_r/LConn2
  b2s q4/RConn1 -- yumi_joint_3_r/LConn2
  b2s q5/RConn1 -- yumi_joint_4_r/LConn2
  b2s q6/RConn1 -- yumi_joint_5_r/LConn2
  b2s q7/RConn1 -- yumi_joint_6_r/LConn2
  yumi_joint_1_r/RConn2 -- q_sensor_1/LConn1
  yumi_joint_1_r/RConn3 -- dq_sensor_1/LConn1
  yumi_joint_2_r/RConn2 -- q_sensor_2/LConn1
  yumi_joint_2_r/RConn3 -- dq_sensor_2/LConn1
  yumi_joint_7_r/RConn2 -- q_sensor_3/LConn1
  yumi_joint_7_r/RConn3 -- dq_sensor_3/LConn1
  yumi_joint_3_r/RConn2 -- q_sensor_4/LConn1
  yumi_joint_3_r/RConn3 -- dq_sensor_4/LConn1
  yumi_joint_4_r/RConn2 -- q_sensor_5/LConn1
  yumi_joint_4_r/RConn3 -- dq_sensor_5/LConn1
  yumi_joint_5_r/RConn2 -- q_sensor_6/LConn1
  yumi_joint_5_r/RConn3 -- dq_sensor_6/LConn1
  yumi_joint_6_r/RConn2 -- q_sensor_7/LConn1
  yumi_joint_6_r/RConn3 -- dq_sensor_7/LConn1
  Simulink-PS Converter/RConn1 -- gripper_r_joint/LConn2

== system XROBO02_reference/Robot/Block 1 ==
  Brick Solid : sm_lib/Body Elements/Brick Solid  BrickDimensions=[1 1 1]*cube_l  BrickDimensionsUnits=m  ExportEntireGeometry=on  InertiaType=CalculateFromGeometry  BasedOnType=Density  Density=1000  DensityUnits=kg/m^3  Mass=1  MassUnits=kg  CenterOfMass=[0 0 0]  CenterOfMassUnits=m  MomentsOfInertia=[1 1 1]  MomentsOfInertiaUnits=kg*m^2  ProductsOfInertia=[0 0 0]  ProductsOfInertiaUnits=kg*m^2  GraphicType=FromGeometry  MarkerShape=Sphere  MarkerSize=10  GraphicVisPropType=SimpleVisualProperties  GraphicDiffuseColor=[1.0 0.6 0.0]  GraphicOpacity=1.0  GraphicSpecularColor=[0.5 0.5 0.5 1.0]  GraphicAmbientColor=[0.15 0.15 0.15 1.0]  GraphicEmissiveColor=[0.0 0.0 0.0 1.0]  GraphicShininess=75  DoExposeReferenceFrame=on  SerializedFrames=<Frames/>
  Point Cloud : sm_lib/Curves and Surfaces/Point Cloud  CoordinatesMatrix=brick_point_cloud  CoordinatesMatrixUnits=m  GraphicType=MarkerCloud  GraphicSphereRadius=1e-3  GraphicSphereRadiusUnits=m  GraphicVisPropType=SimpleVisualProperties  GraphicDiffuseColor=[1 0 0]  GraphicOpacity=1.0  GraphicSpecularColor=[0.5 0.5 0.5 1.0]  GraphicAmbientColor=[0.15 0.15 0.15 1.0]  GraphicEmissiveColor=[0.0 0.0 0.0 1.0]  GraphicShininess=75
  G : PMIOPort  Side=Left
  R : PMIOPort  Port=2  Side=Right
  C : PMIOPort  Port=3  Side=Left
  connections:
  C/RConn1 -- Point Cloud/RConn1
  Point Cloud/LConn1 -- Brick Solid/RConn1 -- R/RConn1
  G/RConn1 -- Brick Solid/LConn1

== system XROBO02_reference/Robot/Block 2 ==
  Brick Solid : sm_lib/Body Elements/Brick Solid  BrickDimensions=[1 1 1]*cube_l  BrickDimensionsUnits=m  ExportEntireGeometry=on  InertiaType=CalculateFromGeometry  BasedOnType=Density  Density=1000  DensityUnits=kg/m^3  Mass=1  MassUnits=kg  CenterOfMass=[0 0 0]  CenterOfMassUnits=m  MomentsOfInertia=[1 1 1]  MomentsOfInertiaUnits=kg*m^2  ProductsOfInertia=[0 0 0]  ProductsOfInertiaUnits=kg*m^2  GraphicType=FromGeometry  MarkerShape=Sphere  MarkerSize=10  GraphicVisPropType=SimpleVisualProperties  GraphicDiffuseColor=[0.0 0.8 0.4]  GraphicOpacity=1.0  GraphicSpecularColor=[0.5 0.5 0.5 1.0]  GraphicAmbientColor=[0.15 0.15 0.15 1.0]  GraphicEmissiveColor=[0.0 0.0 0.0 1.0]  GraphicShininess=75  DoExposeReferenceFrame=on  SerializedFrames=<Frames/>
  Point Cloud : sm_lib/Curves and Surfaces/Point Cloud  CoordinatesMatrix=brick_point_cloud  CoordinatesMatrixUnits=m  GraphicType=MarkerCloud  GraphicSphereRadius=1e-3  GraphicSphereRadiusUnits=m  GraphicVisPropType=SimpleVisualProperties  GraphicDiffuseColor=[1 0 0]  GraphicOpacity=1.0  GraphicSpecularColor=[0.5 0.5 0.5 1.0]  GraphicAmbientColor=[0.15 0.15 0.15 1.0]  GraphicEmissiveColor=[0.0 0.0 0.0 1.0]  GraphicShininess=75
  R : PMIOPort  Side=Right
  G : PMIOPort  Port=2  Side=Left
  C : PMIOPort  Port=3  Side=Left
  connections:
  G/RConn1 -- Brick Solid/LConn1
  R/RConn1 -- Brick Solid/RConn1 -- Point Cloud/LConn1
  C/RConn1 -- Point Cloud/RConn1

== system XROBO02_reference/Robot/Body ==
  yumi_base_link : Subsystem
  yumi_base_link_to_body : sm_lib/Joints/Weld Joint  JointMode=Normal  CompositeWrenchDir=FollowerOnBase  CompositeWrenchFrame=BaseFrame  SenseConstraintForce=off  SenseConstraintTorque=off  SenseTotalForce=off  SenseTotalTorque=off
  yumi_body : Subsystem
  F1 : PMIOPort  Side=Right
  F2 : PMIOPort  Port=2  Side=Right
  F : PMIOPort  Port=3  Side=Left
  connections:
  yumi_base_link/RConn1 -- yumi_base_link_to_body/LConn1
  yumi_base_link_to_body/RConn1 -- yumi_body/LConn1
  yumi_base_link/LConn1 -- F/RConn1
  yumi_body/RConn1 -- F1/RConn1
  yumi_body/RConn2 -- F2/RConn1

== system XROBO02_reference/Robot/Floor ==
  Brick Solid : sm_lib/Body Elements/Brick Solid  BrickDimensions=[1 1 0.01]  BrickDimensionsUnits=m  ExportEntireGeometry=off  InertiaType=CalculateFromGeometry  BasedOnType=Density  Density=1000  DensityUnits=kg/m^3  Mass=1  MassUnits=kg  CenterOfMass=[0 0 0]  CenterOfMassUnits=m  MomentsOfInertia=[1 1 1]  MomentsOfInertiaUnits=kg*m^2  ProductsOfInertia=[0 0 0]  ProductsOfInertiaUnits=kg*m^2  GraphicType=FromGeometry  MarkerShape=Sphere  MarkerSize=10  GraphicVisPropType=SimpleVisualProperties  GraphicDiffuseColor=[0.5 0.5 0.5]  GraphicOpacity=1.0  GraphicSpecularColor=[0.5 0.5 0.5 1.0]  GraphicAmbientColor=[0.15 0.15 0.15 1.0]  GraphicEmissiveColor=[0.0 0.0 0.0 1.0]  GraphicShininess=75  DoExposeReferenceFrame=on  SerializedFrames=<Frames/>
  Rigid Transform : sm_lib/Frames and Transforms/Rigid Transform  RotationMethod=None  FollAlignAxisA=+X  BaseAlignAxisA=+Y  FollAlignAxisB=+Y  BaseAlignAxisB=+Z  RotationStandardAxis=+Z  RotationAngle=0.0  RotationAngleUnits=deg  RotationArbitraryAxis=[0 0 1]  RotationSequenceAxes=FollowerAxes  RotationSequence=XYX  RotationSequenceAngles=[0 0 0]  RotationSequenceAnglesUnits=deg  RotationMatrix=[1 0 0; 0 1 0; 0 0 1]  Quaternion=[1 0 0 0]  TranslationMethod=StandardAxis  TranslationCartesianOffset=[0 0 0]  TranslationCartesianOffsetUnits=m  TranslationStandardAxis=+Z  TranslationStandardOffset=-0.005  TranslationStandardOffsetUnits=m  TranslationROffset=0  TranslationROffsetUnits=m  TranslationThetaOffset=0  TranslationThetaOffsetUnits=deg  TranslationZOffset=0  TranslationZOffsetUnits=m
  T : PMIOPort  Side=Left
  connections:
  Brick Solid/RConn1 -- Rigid Transform/RConn1
  Rigid Transform/LConn1 -- T/RConn1

== system XROBO02_reference/Robot/Arm L/b2s q1 ==
  tau : Inport
  tau_to_ps : nesl_utility/Simulink-PS Converter  PhysicalDomain=network_engine_domain  SubClassName=ps_input  LeftPortType=input  RightPortType=output  PseudoPeriodic=off  Frequencies=[]  NoiseDistribution=none  NoiseParameters=[]  Unit=N*m  AffineConversion=off  FilteringAndDerivatives=provide  SimscapeFilterOrder=1  InputFilterTimeConstant=0.001  UdotUserProvided=0
  s : PMIOPort  Side=Right
  wires:
  tau/1 -> tau_to_ps/1
  connections:
  tau_to_ps/RConn1 -- s/RConn1

== system XROBO02_reference/Robot/Arm L/b2s q2 ==
  tau : Inport
  tau_to_ps : nesl_utility/Simulink-PS Converter  PhysicalDomain=network_engine_domain  SubClassName=ps_input  LeftPortType=input  RightPortType=output  PseudoPeriodic=off  Frequencies=[]  NoiseDistribution=none  NoiseParameters=[]  Unit=N*m  AffineConversion=off  FilteringAndDerivatives=provide  SimscapeFilterOrder=1  InputFilterTimeConstant=0.001  UdotUserProvided=0
  s : PMIOPort  Side=Right
  wires:
  tau/1 -> tau_to_ps/1
  connections:
  tau_to_ps/RConn1 -- s/RConn1

== system XROBO02_reference/Robot/Arm L/b2s q3 ==
  tau : Inport
  tau_to_ps : nesl_utility/Simulink-PS Converter  PhysicalDomain=network_engine_domain  SubClassName=ps_input  LeftPortType=input  RightPortType=output  PseudoPeriodic=off  Frequencies=[]  NoiseDistribution=none  NoiseParameters=[]  Unit=N*m  AffineConversion=off  FilteringAndDerivatives=provide  SimscapeFilterOrder=1  InputFilterTimeConstant=0.001  UdotUserProvided=0
  s : PMIOPort  Side=Right
  wires:
  tau/1 -> tau_to_ps/1
  connections:
  tau_to_ps/RConn1 -- s/RConn1

== system XROBO02_reference/Robot/Arm L/b2s q4 ==
  tau : Inport
  tau_to_ps : nesl_utility/Simulink-PS Converter  PhysicalDomain=network_engine_domain  SubClassName=ps_input  LeftPortType=input  RightPortType=output  PseudoPeriodic=off  Frequencies=[]  NoiseDistribution=none  NoiseParameters=[]  Unit=N*m  AffineConversion=off  FilteringAndDerivatives=provide  SimscapeFilterOrder=1  InputFilterTimeConstant=0.001  UdotUserProvided=0
  s : PMIOPort  Side=Right
  wires:
  tau/1 -> tau_to_ps/1
  connections:
  tau_to_ps/RConn1 -- s/RConn1

== system XROBO02_reference/Robot/Arm L/b2s q5 ==
  tau : Inport
  tau_to_ps : nesl_utility/Simulink-PS Converter  PhysicalDomain=network_engine_domain  SubClassName=ps_input  LeftPortType=input  RightPortType=output  PseudoPeriodic=off  Frequencies=[]  NoiseDistribution=none  NoiseParameters=[]  Unit=N*m  AffineConversion=off  FilteringAndDerivatives=provide  SimscapeFilterOrder=1  InputFilterTimeConstant=0.001  UdotUserProvided=0
  s : PMIOPort  Side=Right
  wires:
  tau/1 -> tau_to_ps/1
  connections:
  tau_to_ps/RConn1 -- s/RConn1

== system XROBO02_reference/Robot/Arm L/b2s q6 ==
  tau : Inport
  tau_to_ps : nesl_utility/Simulink-PS Converter  PhysicalDomain=network_engine_domain  SubClassName=ps_input  LeftPortType=input  RightPortType=output  PseudoPeriodic=off  Frequencies=[]  NoiseDistribution=none  NoiseParameters=[]  Unit=N*m  AffineConversion=off  FilteringAndDerivatives=provide  SimscapeFilterOrder=1  InputFilterTimeConstant=0.001  UdotUserProvided=0
  s : PMIOPort  Side=Right
  wires:
  tau/1 -> tau_to_ps/1
  connections:
  tau_to_ps/RConn1 -- s/RConn1

== system XROBO02_reference/Robot/Arm L/b2s q7 ==
  tau : Inport
  tau_to_ps : nesl_utility/Simulink-PS Converter  PhysicalDomain=network_engine_domain  SubClassName=ps_input  LeftPortType=input  RightPortType=output  PseudoPeriodic=off  Frequencies=[]  NoiseDistribution=none  NoiseParameters=[]  Unit=N*m  AffineConversion=off  FilteringAndDerivatives=provide  SimscapeFilterOrder=1  InputFilterTimeConstant=0.001  UdotUserProvided=0
  s : PMIOPort  Side=Right
  wires:
  tau/1 -> tau_to_ps/1
  connections:
  tau_to_ps/RConn1 -- s/RConn1
